simulink model "soft_robot_model_with_revolute_joints"  (R2025b)
settings: Solver=VariableStepAuto  StartTime=0.0  StopTime=5.0  RelTol=1e-3
values from neighbouring files (symbols this model uses):
  d_z = 0    [Code4Simulink.m]
  L = 0.15    [Code4Simulink.m]
  phi = [30, 150, 270] * pi/180    [Code4Simulink.m]
  theta_x = deg2rad(0)    [Code4Simulink.m]
  theta_y = deg2rad(0)    [Code4Simulink.m]
undefined symbols (not defined in the file or in its folder): X, Y, Z
libraries: sm_lib x29, nesl_utility x4
(part 2 of 2)

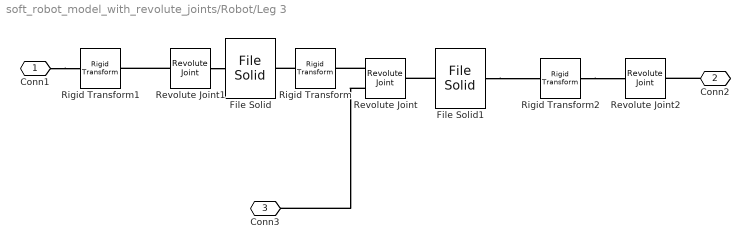
== system soft_robot_model_with_revolute_joints/Robot/Leg 3 ==
  File Solid : sm_lib/Body Elements/File Solid  ExtGeomFileName=/Users/didar/Downloads/Side_Link.STEP  UnitType=FromFile  ExtGeomFileUnits=m  StepReaderType=HEX  ExportConvexHullGeometry=off  InertiaType=Custom  BasedOnType=DensityFromFile  Density=1000  DensityUnits=kg/m^3  Mass=30  MassUnits=g  CenterOfMass=[0 0 0]  CenterOfMassUnits=m  MomentsOfInertia=[1 1 1]  MomentsOfInertiaUnits=kg*m^2  ProductsOfInertia=[0 0 0]  ProductsOfInertiaUnits=kg*m^2  GraphicType=FromGeometry  MarkerShape=Sphere  MarkerSize=10  GraphicVisPropType=SimpleVisualProperties  GraphicDiffuseColor=[0.5 0.5 0.5]  GraphicOpacity=1  GraphicSpecularColor=[0.5 0.5 0.5 1.0]  GraphicAmbientColor=[0.15 0.15 0.15 1.0]  GraphicEmissiveColor=[0.0 0.0 0.0 1.0]  GraphicShininess=75  DoExposeReferenceFrame=off  SerializedFrames=|
      | <Frames>
      | 
      |   <Frame>
      |     <Id>Frame1</Id>
      |     <Value>
      |       <Name>F</Name>
      |       <Origin>
      |         <Source>GeometricFeature</Source>
      |         <FeatureName>planar surface 8</FeatureName>
      |       </Origin>
      |       <PrimaryAxis>
      |         <DefinedDirection>+Z</DefinedDirection>
      |         <Source>ReferenceFrame</Source>
      |         <SourceDirection>+Z</SourceDirection>
      |         <FeatureName></FeatureName>
      |       </PrimaryAxis>
      |       <SecondaryAxis>
      |         <DefinedDirection>+X</DefinedDirection>
      |         <Source>GeometricFeature</Source>
      |         <SourceDirection>+X</SourceDirection>
      |         <FeatureName>planar surface 11</FeatureName>
      |       </SecondaryAxis>
      |     </Value>
      |   </Frame>
      | 
      |   <Frame>
      |     <Id>Frame2</Id>
      |     <Value>
      |       <Name>B</Name>
      |       <Origin>
      |         <Source>GeometricFeature</Source>
      |         <FeatureName>planar surface 5</FeatureName>
      |       </Origin>
      |       <PrimaryAxis>
      |         <DefinedDirection>+Z</DefinedDirection>
      |         <Source>ReferenceFrame</Source>
      |         <SourceDirection>+Z</SourceDirection>
      |         <FeatureName></FeatureName>
      |       </PrimaryAxis>
      |       <SecondaryAxis>
      |         <DefinedDirection>+X</DefinedDirection>
      |         <Source>GeometricFeature</Source>
      |         <SourceDirection>+X</SourceDirection>
      |         <FeatureName>planar surface 3</FeatureName>
      |       </SecondaryAxis>
      |     </Value>
      |   </Frame>
      | 
      | </Frames>
  File Solid1 : sm_lib/Body Elements/File Solid  ExtGeomFileName=/Users/didar/Downloads/Side_Link.STEP  UnitType=FromFile  ExtGeomFileUnits=m  StepReaderType=HEX  ExportConvexHullGeometry=off  InertiaType=Custom  BasedOnType=DensityFromFile  Density=1000  DensityUnits=kg/m^3  Mass=30  MassUnits=g  CenterOfMass=[0 0 0]  CenterOfMassUnits=m  MomentsOfInertia=[1 1 1]  MomentsOfInertiaUnits=kg*m^2  ProductsOfInertia=[0 0 0]  ProductsOfInertiaUnits=kg*m^2  GraphicType=FromGeometry  MarkerShape=Sphere  MarkerSize=10  GraphicVisPropType=SimpleVisualProperties  GraphicDiffuseColor=[0.5 0.5 0.5]  GraphicOpacity=1  GraphicSpecularColor=[0.5 0.5 0.5 1.0]  GraphicAmbientColor=[0.15 0.15 0.15 1.0]  GraphicEmissiveColor=[0.0 0.0 0.0 1.0]  GraphicShininess=75  DoExposeReferenceFrame=off  SerializedFrames=|
      | <Frames>
      | 
      |   <Frame>
      |     <Id>Frame1</Id>
      |     <Value>
      |       <Name>F</Name>
      |       <Origin>
      |         <Source>GeometricFeature</Source>
      |         <FeatureName>planar surface 8</FeatureName>
      |       </Origin>
      |       <PrimaryAxis>
      |         <DefinedDirection>+Z</DefinedDirection>
      |         <Source>ReferenceFrame</Source>
      |         <SourceDirection>+Z</SourceDirection>
      |         <FeatureName></FeatureName>
      |       </PrimaryAxis>
      |       <SecondaryAxis>
      |         <DefinedDirection>+X</DefinedDirection>
      |         <Source>GeometricFeature</Source>
      |         <SourceDirection>+X</SourceDirection>
      |         <FeatureName>planar surface 11</FeatureName>
      |       </SecondaryAxis>
      |     </Value>
      |   </Frame>
      | 
      |   <Frame>
      |     <Id>Frame2</Id>
      |     <Value>
      |       <Name>B</Name>
      |       <Origin>
      |         <Source>GeometricFeature</Source>
      |         <FeatureName>planar surface 5</FeatureName>
      |       </Origin>
      |       <PrimaryAxis>
      |         <DefinedDirection>+Z</DefinedDirection>
      |         <Source>ReferenceFrame</Source>
      |         <SourceDirection>+Z</SourceDirection>
      |         <FeatureName></FeatureName>
      |       </PrimaryAxis>
      |       <SecondaryAxis>
      |         <DefinedDirection>+X</DefinedDirection>
      |         <Source>GeometricFeature</Source>
      |         <SourceDirection>+X</SourceDirection>
      |         <FeatureName>planar surface 3</FeatureName>
      |       </SecondaryAxis>
      |     </Value>
      |   </Frame>
      | 
      | </Frames>
  Revolute Joint : sm_lib/Joints/Revolute Joint  JointMode=Normal  CompositeWrenchDir=FollowerOnBase  CompositeWrenchFrame=BaseFrame  SenseConstraintForce=off  SenseConstraintTorque=off  SenseTotalForce=off  SenseTotalTorque=off  PositionTargetSpecify=off  PositionTargetPriority=High  PositionTargetValue=0  PositionTargetValueUnits=deg  VelocityTargetSpecify=off  VelocityTargetPriority=High  VelocityTargetValue=0  VelocityTargetValueUnits=deg/s  EquilibriumPosition=0  EquilibriumPositionUnits=deg  SpringStiffness=0.5  SpringStiffnessUnits=N*m/deg  DampingCoefficient=0.2  DampingCoefficientUnits=N*m/(deg/s)  LowerLimitSpecify=off  LowerLimitBound=-90  LowerLimitBoundUnits=deg  LowerLimitStiffness=1e4  LowerLimitStiffnessUnits=N*m/deg  LowerLimitDamping=10  LowerLimitDampingUnits=N*m/(deg/s)  LowerLimitTransitionRegionWidth=0.1  LowerLimitTransitionRegionWidthUnits=deg  UpperLimitSpecify=off  UpperLimitBound=90  UpperLimitBoundUnits=deg  UpperLimitStiffness=1e4  UpperLimitStiffnessUnits=N*m/deg  UpperLimitDamping=10  UpperLimitDampingUnits=N*m/(deg/s)  UpperLimitTransitionRegionWidth=0.1  UpperLimitTransitionRegionWidthUnits=deg  TorqueActuationMode=InputTorque  MotionActuationMode=ComputedMotion  SensePosition=off  SenseVelocity=off  SenseAcceleration=off  SenseTorqueForce=off  SenseLowerLimitTorqueForce=off  SenseUpperLimitTorqueForce=off
  Revolute Joint1 : sm_lib/Joints/Revolute Joint  JointMode=Normal  CompositeWrenchDir=FollowerOnBase  CompositeWrenchFrame=BaseFrame  SenseConstraintForce=off  SenseConstraintTorque=off  SenseTotalForce=off  SenseTotalTorque=off  PositionTargetSpecify=off  PositionTargetPriority=High  PositionTargetValue=0  PositionTargetValueUnits=deg  VelocityTargetSpecify=off  VelocityTargetPriority=High  VelocityTargetValue=0  VelocityTargetValueUnits=deg/s  EquilibriumPosition=0  EquilibriumPositionUnits=deg  SpringStiffness=0.5  SpringStiffnessUnits=N*m/deg  DampingCoefficient=0.2  DampingCoefficientUnits=N*m/(deg/s)  LowerLimitSpecify=off  LowerLimitBound=-90  LowerLimitBoundUnits=deg  LowerLimitStiffness=1e4  LowerLimitStiffnessUnits=N*m/deg  LowerLimitDamping=10  LowerLimitDampingUnits=N*m/(deg/s)  LowerLimitTransitionRegionWidth=0.1  LowerLimitTransitionRegionWidthUnits=deg  UpperLimitSpecify=off  UpperLimitBound=90  UpperLimitBoundUnits=deg  UpperLimitStiffness=1e4  UpperLimitStiffnessUnits=N*m/deg  UpperLimitDamping=10  UpperLimitDampingUnits=N*m/(deg/s)  UpperLimitTransitionRegionWidth=0.1  UpperLimitTransitionRegionWidthUnits=deg  TorqueActuationMode=NoTorque  MotionActuationMode=ComputedMotion  SensePosition=off  SenseVelocity=off  SenseAcceleration=off  SenseTorqueForce=off  SenseLowerLimitTorqueForce=off  SenseUpperLimitTorqueForce=off
  Revolute Joint2 : sm_lib/Joints/Revolute Joint  JointMode=Normal  CompositeWrenchDir=FollowerOnBase  CompositeWrenchFrame=BaseFrame  SenseConstraintForce=off  SenseConstraintTorque=off  SenseTotalForce=off  SenseTotalTorque=off  PositionTargetSpecify=off  PositionTargetPriority=High  PositionTargetValue=0  PositionTargetValueUnits=deg  VelocityTargetSpecify=off  VelocityTargetPriority=High  VelocityTargetValue=0  VelocityTargetValueUnits=deg/s  EquilibriumPosition=0  EquilibriumPositionUnits=deg  SpringStiffness=0.5  SpringStiffnessUnits=N*m/deg  DampingCoefficient=0.2  DampingCoefficientUnits=N*m/(deg/s)  LowerLimitSpecify=off  LowerLimitBound=-90  LowerLimitBoundUnits=deg  LowerLimitStiffness=1e4  LowerLimitStiffnessUnits=N*m/deg  LowerLimitDamping=10  LowerLimitDampingUnits=N*m/(deg/s)  LowerLimitTransitionRegionWidth=0.1  LowerLimitTransitionRegionWidthUnits=deg  UpperLimitSpecify=off  UpperLimitBound=90  UpperLimitBoundUnits=deg  UpperLimitStiffness=1e4  UpperLimitStiffnessUnits=N*m/deg  UpperLimitDamping=10  UpperLimitDampingUnits=N*m/(deg/s)  UpperLimitTransitionRegionWidth=0.1  UpperLimitTransitionRegionWidthUnits=deg  TorqueActuationMode=NoTorque  MotionActuationMode=ComputedMotion  SensePosition=off  SenseVelocity=off  SenseAcceleration=off  SenseTorqueForce=off  SenseLowerLimitTorqueForce=off  SenseUpperLimitTorqueForce=off
  Rigid Transform : sm_lib/Frames and Transforms/Rigid Transform  RotationMethod=StandardAxis  FollAlignAxisA=+X  BaseAlignAxisA=+Y  FollAlignAxisB=+Y  BaseAlignAxisB=+Z  RotationStandardAxis=+Z  RotationAngle=60  RotationAngleUnits=deg  RotationArbitraryAxis=[0 0 1]  RotationSequenceAxes=FollowerAxes  RotationSequence=XYX  RotationSequenceAngles=[0 0 0]  RotationSequenceAnglesUnits=deg  RotationMatrix=[1 0 0;0 1 0;0 0 1]  Quaternion=[1 0 0 0]  TranslationMethod=Cartesian  TranslationCartesianOffset=[1 -2 0]  TranslationCartesianOffsetUnits=cm  TranslationStandardAxis=+Z  TranslationStandardOffset=0  TranslationStandardOffsetUnits=m  TranslationROffset=0  TranslationROffsetUnits=m  TranslationThetaOffset=0  TranslationThetaOffsetUnits=deg  TranslationZOffset=0  TranslationZOffsetUnits=m
  Rigid Transform1 : sm_lib/Frames and Transforms/Rigid Transform  RotationMethod=StandardAxis  FollAlignAxisA=+X  BaseAlignAxisA=+Y  FollAlignAxisB=+Y  BaseAlignAxisB=+Z  RotationStandardAxis=+Z  RotationAngle=-30  RotationAngleUnits=deg  RotationArbitraryAxis=[0 0 1]  RotationSequenceAxes=FollowerAxes  RotationSequence=XYX  RotationSequenceAngles=[0 0 0]  RotationSequenceAnglesUnits=deg  RotationMatrix=[1 0 0;0 1 0;0 0 1]  Quaternion=[1 0 0 0]  TranslationMethod=Cartesian  TranslationCartesianOffset=[-2 -1 0]  TranslationCartesianOffsetUnits=cm  TranslationStandardAxis=+Z  TranslationStandardOffset=0  TranslationStandardOffsetUnits=m  TranslationROffset=0  TranslationROffsetUnits=m  TranslationThetaOffset=0  TranslationThetaOffsetUnits=deg  TranslationZOffset=0  TranslationZOffsetUnits=m
  Rigid Transform2 : sm_lib/Frames and Transforms/Rigid Transform  RotationMethod=StandardAxis  FollAlignAxisA=+X  BaseAlignAxisA=+Y  FollAlignAxisB=+Y  BaseAlignAxisB=+Z  RotationStandardAxis=+Z  RotationAngle=-30  RotationAngleUnits=deg  RotationArbitraryAxis=[0 0 1]  RotationSequenceAxes=FollowerAxes  RotationSequence=XYX  RotationSequenceAngles=[0 0 0]  RotationSequenceAnglesUnits=deg  RotationMatrix=[1 0 0;0 1 0;0 0 1]  Quaternion=[1 0 0 0]  TranslationMethod=Cartesian  TranslationCartesianOffset=[1 -2 0]  TranslationCartesianOffsetUnits=cm  TranslationStandardAxis=+Z  TranslationStandardOffset=0  TranslationStandardOffsetUnits=m  TranslationROffset=0  TranslationROffsetUnits=m  TranslationThetaOffset=0  TranslationThetaOffsetUnits=deg  TranslationZOffset=0  TranslationZOffsetUnits=m
  Conn1 : PMIOPort  Side=Left
  Conn2 : PMIOPort  Port=2  Side=Right
  Conn3 : PMIOPort  Port=3  Side=Left
  connections:
  Conn2/RConn1 -- Revolute Joint2/RConn1
  Revolute Joint1/LConn1 -- Rigid Transform1/RConn1
  Conn1/RConn1 -- Rigid Transform1/LConn1
  File Solid1/RConn1 -- Revolute Joint/RConn1
  Rigid Transform/LConn1 -- File Solid/LConn1
  Rigid Transform2/RConn1 -- Revolute Joint2/LConn1
  Revolute Joint/LConn1 -- Rigid Transform/RConn1
  Revolute Joint/LConn2 -- Conn3/RConn1
  Revolute Joint1/RConn1 -- File Solid/RConn1
  File Solid1/LConn1 -- Rigid Transform2/LConn1

== matlab function soft_robot_model_with_revolute_joints/MATLAB Function ==
  data: theta_x input; beta1 output; theta_y input; d_z input; L input; phi input; beta2 output; beta3 output
function [beta1, beta2, beta3] = kinematics(theta_x, theta_y, d_z, L, phi)
    % Base bending from height
    beta_base = 2 * acos(1 - d_z / (2*L));
    
    % Tilt projection onto each leg
    beta_tilt = theta_x * cos(phi) + theta_y * sin(phi);
    
    % Total bending per leg
    betas = beta_base + beta_tilt;
    
    beta1 = betas(1);
    beta2 = betas(2);
    beta3 = betas(3);
end
